simulink model "servo_identified"  (R2023b)
settings: Solver=ode1  StartTime=0.0  StopTime=Tend  FixedStep=dt  RelTol=1e-3
model workspace (MAT data in the model file):
  K = 1
  Kd = 0
  Ki = 1.5
  KiOn = 1
  Kp = 0.3
  Tend = 5
  Tf = 0.01
  Ts = 0.1
  aTF = 0.990049833749
  acc = 50
  aw = 1
  blWidth = 1e-09
  closedLoop = 1
  dt = 0.001
  dz = 0
  measSel = 1
  nLat = 70
  nTheta = 0
  olProfile = [0 60]
  qCnt = 1
  qSpd = 4.615
  sensorAtLoad = 0
  spProfile = [0 60]
  uMax = 180
undefined symbols (not defined in the file or in its folder): DiscIntNeverNeededParam
libraries: simulink x2
settings Model: Creator=odyssix  LastModifiedBy=odyssix
settings ModelReferenceCC: UpdateModelReferenceTargets=IfOutOfDate
settings RTWCC: GPUComputeCapability=5.0
settings ConfigComp: CovBoundaryAbsTol=1.0e-5

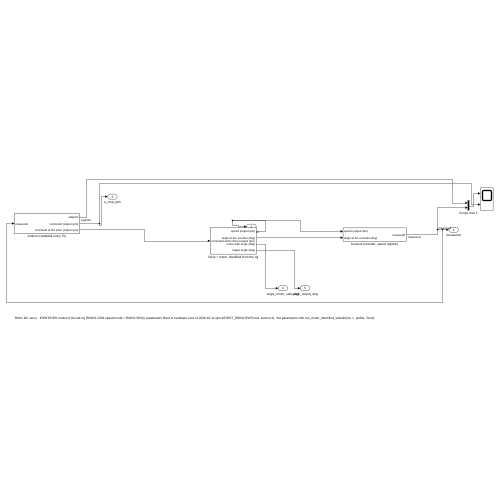
[thumbnail: Simulink's stored preview of the top-level diagram]
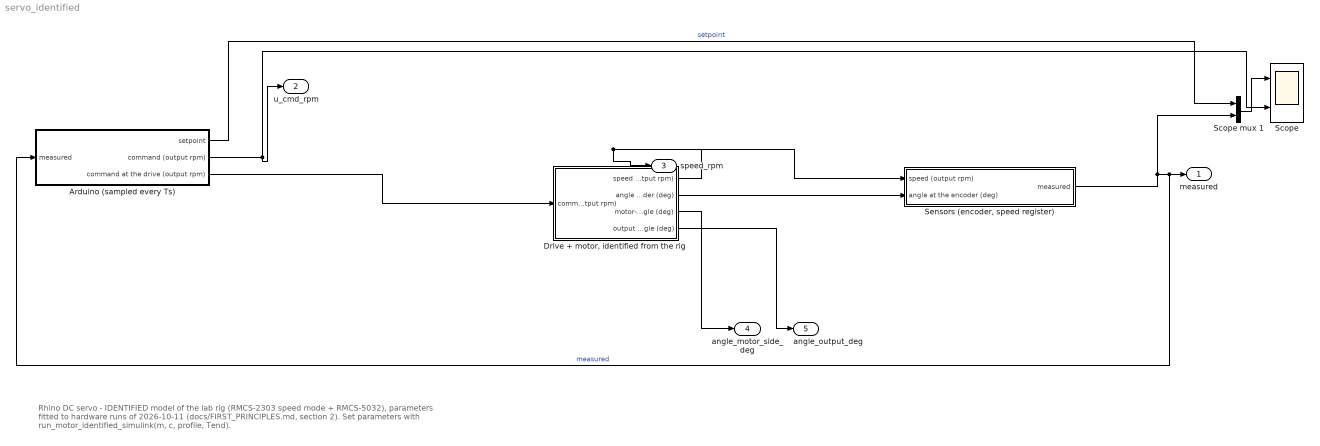
== system servo_identified ==
  note: Rhino DC servo - IDENTIFIED model of the lab rig (RMCS-2303 speed mode + RMCS-5032), parameters fitted to hardware runs of 2026-10-11 (docs/FIRST_PRINCIPLES.md, section 2). Set parameters with run_motor_identified_simulink(m, c, profile, Tend).
  Arduino (sampled every Ts) : Subsystem
  "Drive + motor, identified from the rig" : Subsystem
  Scope : Scope  NumInputPorts=2
  Scope mux 1 : Mux  Inputs=2
  "Sensors (encoder, speed register)" : Subsystem
  measured : Outport
  u_cmd_rpm : Outport  Port=2
  speed_rpm : Outport  Port=3
  angle_motor_side_deg : Outport  Port=4
  angle_output_deg : Outport  Port=5
  wires:
  Scope mux 1/1 -> Scope/1
  Arduino (sampled every Ts)/2(command (output rpm)) -> u_cmd_rpm/1, Scope/2
  Arduino (sampled every Ts)/1(setpoint) -> Scope mux 1/1  "setpoint"
  "Sensors (encoder, speed register)"/1(measured) -> Arduino (sampled every Ts)/1(measured), measured/1, Scope mux 1/2  "measured"
  "Drive + motor, identified from the rig"/1(speed (output rpm)) -> speed_rpm/1, "Sensors (encoder, speed register)"/1(speed (output rpm))
  Arduino (sampled every Ts)/3(command at the drive (output rpm)) -> "Drive + motor, identified from the rig"/1(command at the drive (output rpm))
  "Drive + motor, identified from the rig"/2(angle at the encoder (deg)) -> "Sensors (encoder, speed register)"/2(angle at the encoder (deg))
  "Drive + motor, identified from the rig"/3(motor-side angle (deg)) -> angle_motor_side_deg/1
  "Drive + motor, identified from the rig"/4(output angle (deg)) -> angle_output_deg/1

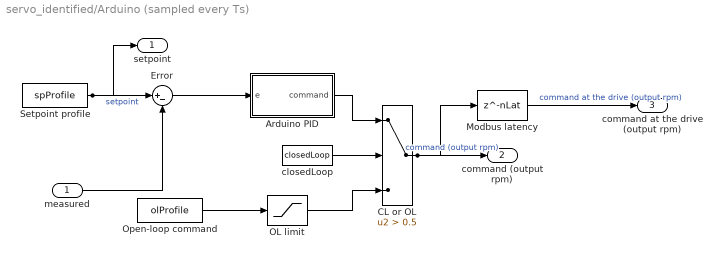
== system servo_identified/Arduino (sampled every Ts) ==
  measured : Inport
  Arduino PID : Subsystem
  CL or OL : Switch  Criteria=u2 > Threshold  Threshold=0.5  SaturateOnIntegerOverflow=off  InputSameDT=off
  Error : Sum  Inputs=|+-
  Modbus latency : Delay  DelayLength=nLat  SampleTime=dt
  OL limit : Saturate  UpperLimit=uMax  LowerLimit=-uMax
  Open-loop command : FromWorkspace  VariableName=olProfile  SampleTime=Ts  Interpolate=off  OutputAfterFinalValue=Holding final value
  Setpoint profile : FromWorkspace  VariableName=spProfile  SampleTime=Ts  Interpolate=off  OutputAfterFinalValue=Holding final value
  closedLoop : Constant  Value=closedLoop
  setpoint : Outport
  command (output rpm) : Outport  Port=2
  command at the drive (output rpm) : Outport  Port=3
  wires:
  CL or OL/1 -> Modbus latency/1, command (output rpm)/1  "command (output rpm)"
  Modbus latency/1 -> command at the drive (output rpm)/1  "command at the drive (output rpm)"
  OL limit/1 -> CL or OL/3
  Arduino PID/1(command) -> CL or OL/1
  closedLoop/1 -> CL or OL/2
  Open-loop command/1 -> OL limit/1
  Error/1 -> Arduino PID/1(e)
  measured/1 -> Error/2
  Setpoint profile/1 -> setpoint/1, Error/1  "setpoint"

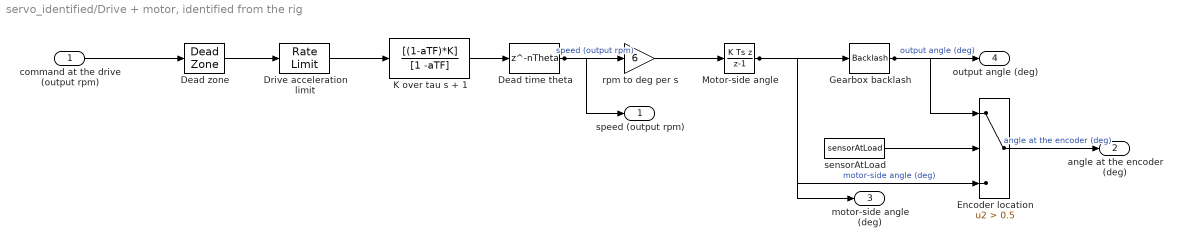
== system servo_identified/Drive + motor, identified from the rig ==
  command at the drive (output rpm) : Inport
  Dead time theta : Delay  DelayLength=nTheta  SampleTime=dt
  Dead zone : DeadZone  LowerValue=-dz  UpperValue=dz
  Drive acceleration limit : RateLimiter  RisingSlewLimit=acc  FallingSlewLimit=-acc  SampleTimeMode=inherited
  Encoder location : Switch  Criteria=u2 > Threshold  Threshold=0.5  SaturateOnIntegerOverflow=off  InputSameDT=off
  Gearbox backlash : Backlash  BacklashWidth=blWidth
  K over tau s + 1 : DiscreteTransferFcn  Numerator=[(1-aTF)*K]  Denominator=[1 -aTF]  SampleTime=dt
  Motor-side angle : DiscreteIntegrator  IntegratorMethod=Integration: Backward Euler  SampleTime=dt  ICPrevOutput=DiscIntNeverNeededParam  ICPrevScaledInput=DiscIntNeverNeededParam
  rpm to deg per s : Gain  Gain=6
  sensorAtLoad : Constant  Value=sensorAtLoad
  speed (output rpm) : Outport
  angle at the encoder (deg) : Outport  Port=2
  motor-side angle (deg) : Outport  Port=3
  output angle (deg) : Outport  Port=4
  wires:
  Dead time theta/1 -> rpm to deg per s/1, speed (output rpm)/1  "speed (output rpm)"
  Encoder location/1 -> angle at the encoder (deg)/1  "angle at the encoder (deg)"
  Gearbox backlash/1 -> output angle (deg)/1, Encoder location/1  "output angle (deg)"
  K over tau s + 1/1 -> Dead time theta/1
  Motor-side angle/1 -> Gearbox backlash/1, motor-side angle (deg)/1, Encoder location/3  "motor-side angle (deg)"
  Drive acceleration limit/1 -> K over tau s + 1/1
  Dead zone/1 -> Drive acceleration limit/1
  sensorAtLoad/1 -> Encoder location/2
  rpm to deg per s/1 -> Motor-side angle/1
  command at the drive (output rpm)/1 -> Dead zone/1

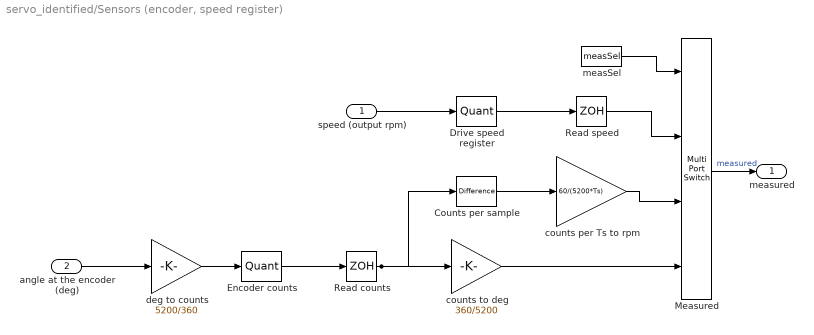
== system servo_identified/Sensors (encoder, speed register) ==
  speed (output rpm) : Inport
  angle at the encoder (deg) : Inport  Port=2
  Counts per sample : simulink/Discrete/Difference  ICPrevInput=0.0  OutMin=[]  OutMax=[]  OutDataType=fixdt(1, 16)  OutScaling=2^-10  DoSatur=off
  Drive speed register : Quantizer  QuantizationInterval=qSpd
  Encoder counts : Quantizer  QuantizationInterval=qCnt
  Measured : MultiPortSwitch  SaturateOnIntegerOverflow=off  InputSameDT=off
  Read counts : ZeroOrderHold  SampleTime=Ts
  Read speed : ZeroOrderHold  SampleTime=Ts
  counts per Ts to rpm : Gain  Gain=60/(5200*Ts)
  counts to deg : Gain  Gain=360/5200
  deg to counts : Gain  Gain=5200/360
  measSel : Constant  Value=measSel
  measured : Outport
  wires:
  Measured/1 -> measured/1  "measured"
  measSel/1 -> Measured/1
  counts to deg/1 -> Measured/4
  Counts per sample/1 -> counts per Ts to rpm/1
  Read speed/1 -> Measured/2
  Drive speed register/1 -> Read speed/1
  counts per Ts to rpm/1 -> Measured/3
  speed (output rpm)/1 -> Drive speed register/1
  Encoder counts/1 -> Read counts/1
  Read counts/1 -> counts to deg/1, Counts per sample/1
  deg to counts/1 -> Encoder counts/1
  angle at the encoder (deg)/1 -> deg to counts/1

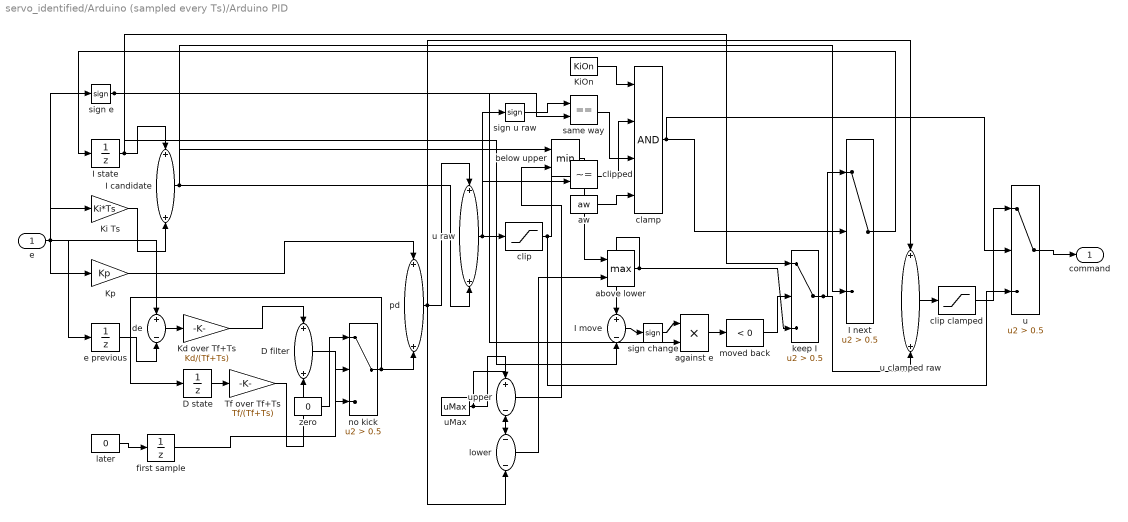
== system servo_identified/Arduino (sampled every Ts)/Arduino PID ==
  e : Inport
  D filter : Sum
  D state : UnitDelay  SampleTime=Ts
  I candidate : Sum
  I move : Sum  Inputs=+-
  I next : Switch  Criteria=u2 > Threshold  Threshold=0.5  SaturateOnIntegerOverflow=off  InputSameDT=off
  I state : UnitDelay  SampleTime=Ts
  Kd over Tf+Ts : Gain  Gain=Kd/(Tf+Ts)
  Ki Ts : Gain  Gain=Ki*Ts
  KiOn : Constant  Value=KiOn
  Kp : Gain  Gain=Kp
  Tf over Tf+Ts : Gain  Gain=Tf/(Tf+Ts)
  above lower : MinMax  Function=max  Inputs=2
  against e : Product
  aw : Constant  Value=aw
  below upper : MinMax  Inputs=2
  clamp : Logic  Inputs=4  AllPortsSameDT=off  OutDataTypeStr=boolean
  clip : Saturate  UpperLimit=uMax  LowerLimit=-uMax
  clip clamped : Saturate  UpperLimit=uMax  LowerLimit=-uMax
  clipped : RelationalOperator  Operator=~=  OutDataTypeStr=boolean  RndMeth=Simplest  InputSameDT=off
  de : Sum  Inputs=+-
  e previous : UnitDelay  SampleTime=Ts
  first sample : UnitDelay  InitialCondition=1  SampleTime=Ts
  keep I : Switch  Criteria=u2 > Threshold  Threshold=0.5  SaturateOnIntegerOverflow=off  InputSameDT=off
  later : Constant  Value=0
  lower : Sum  Inputs=--
  moved back : simulink/Logic and Bit Operations/Compare To Constant  relop=<  const=0  OutDataTypeStr=boolean
  no kick : Switch  Criteria=u2 > Threshold  Threshold=0.5  SaturateOnIntegerOverflow=off  InputSameDT=off
  pd : Sum
  same way : RelationalOperator  Operator===  OutDataTypeStr=boolean  RndMeth=Simplest  InputSameDT=off
  sign change : Signum
  sign e : Signum
  sign u raw : Signum
  u : Switch  Criteria=u2 > Threshold  Threshold=0.5  SaturateOnIntegerOverflow=off  InputSameDT=off
  u clamped raw : Sum
  u raw : Sum
  uMax : Constant  Value=uMax
  upper : Sum  Inputs=+-
  zero : Constant  Value=0
  command : Outport
  wires:
  e/1 -> e previous/1, de/1, Ki Ts/1, Kp/1, sign e/1
  e previous/1 -> de/2
  de/1 -> Kd over Tf+Ts/1
  D state/1 -> Tf over Tf+Ts/1
  Kd over Tf+Ts/1 -> D filter/1
  Tf over Tf+Ts/1 -> D filter/2
  later/1 -> first sample/1
  zero/1 -> no kick/1
  first sample/1 -> no kick/2
  D filter/1 -> no kick/3
  no kick/1 -> D state/1, pd/2
  I state/1 -> I candidate/1, I move/2, keep I/1
  Ki Ts/1 -> I candidate/2
  Kp/1 -> pd/1
  pd/1 -> u raw/1, upper/2, lower/2, u clamped raw/1
  I candidate/1 -> u raw/2, below upper/1, I next/3
  u raw/1 -> clip/1, clipped/2, sign u raw/1
  clip/1 -> clipped/1, u/3
  sign u raw/1 -> same way/1
  sign e/1 -> same way/2, against e/2
  KiOn/1 -> clamp/1
  clipped/1 -> clamp/2
  same way/1 -> clamp/3
  aw/1 -> clamp/4
  uMax/1 -> upper/1, lower/1
  upper/1 -> below upper/2
  below upper/1 -> above lower/1
  lower/1 -> above lower/2
  above lower/1 -> I move/1, keep I/3
  I move/1 -> sign change/1
  sign change/1 -> against e/1
  against e/1 -> moved back/1
  moved back/1 -> keep I/2
  keep I/1 -> I next/1, u clamped raw/2
  clamp/1 -> I next/2, u/2
  I next/1 -> I state/1
  u clamped raw/1 -> clip clamped/1
  clip clamped/1 -> u/1
  u/1 -> command/1
